simulink model "shc_heating_cooling"  (R2023a)
settings: Solver=ode4  StartTime=0.0  StopTime=500  FixedStep=0.1  RelTol=1e-3
model workspace (MAT data in the model file):
  A_demo = 0.5
  P_demo = 100
  T0_demo = 20
  Tenv_demo = 20
  cp_demo = 1000
  h_demo = 10
  mass_demo = 0.5
libraries: SHCLib x4
settings Model: Creator=hwx20  LastModifiedBy=hwx20

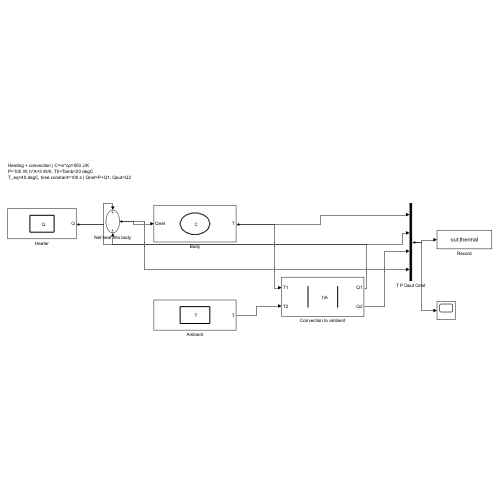
[thumbnail: Simulink's stored preview of the top-level diagram]
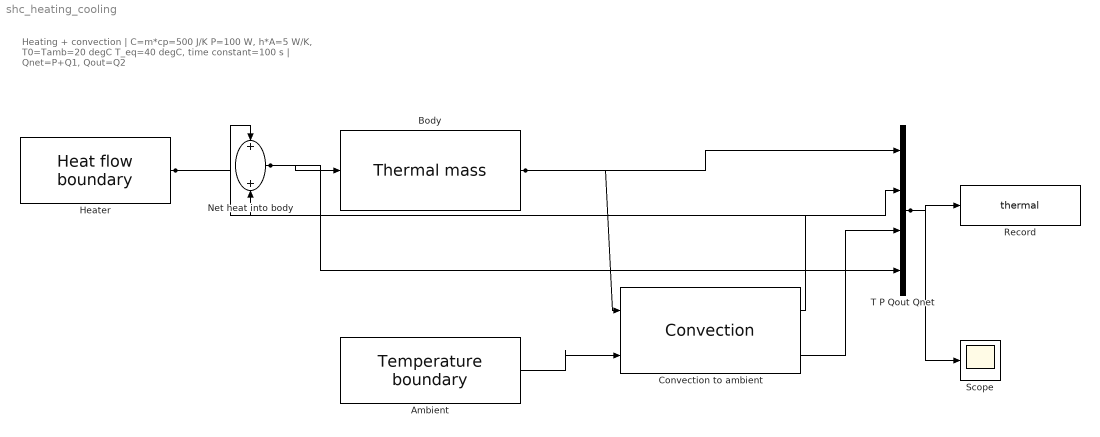
== system shc_heating_cooling ==
  note: Heating + convection | C=m*cp=500 J/K
      | P=100 W, h*A=5 W/K, T0=Tamb=20 degC
      | T_eq=40 degC, time constant=100 s | Qnet=P+Q1, Qout=Q2
  Ambient : SHCLib/Temperature boundary  temperature=Tenv_demo
      settings: SourceProductName=Heat Conduction
  Body : SHCLib/Thermal mass  mass=mass_demo  cp=cp_demo  Tinit=T0_demo
      settings: SourceProductName=Heat Conduction
  Convection to ambient : SHCLib/Convection  h=h_demo  area=A_demo
      settings: SourceProductName=Heat Conduction
  Heater : SHCLib/Heat flow boundary  power=P_demo
      settings: SourceProductName=Heat Conduction
  Net heat into body : Sum
  Record : ToWorkspace  VariableName=thermal  SaveFormat=Structure With Time  SampleTime=-1
  Scope : Scope
  T P Qout Qnet : Mux
  wires:
  Heater/1 -> Net heat into body/1, T P Qout Qnet/2
  Convection to ambient/1 -> Net heat into body/2
  Net heat into body/1 -> Body/1, T P Qout Qnet/4
  Body/1 -> Convection to ambient/1, T P Qout Qnet/1
  Ambient/1 -> Convection to ambient/2
  Convection to ambient/2 -> T P Qout Qnet/3
  T P Qout Qnet/1 -> Record/1, Scope/1
